simulink model "afe_dqctrl_inv_psm"  (R2026a)
settings: Solver=ode23t  StopTime=simlength  FixedStep=tc  MaxStep=glb_time.tc  RelTol=1e-4
values from neighbouring files (symbols this model uses):
  afe_ctrl = ctrl_afe_setup(glb_time.ts_afe, grid_emu.omega_grid_nom)    [init_model.m]
  afe_pwm_phase_shift_mod1 = 0    [init_model.m]
  CTRPIFF_CLIP_RELEASE = 0.001    [init_model.m]
  filters = setup_global_filters(glb_time.ts_afe, glb_time.ts_inv, glb_time.ts_dab, glb_time.tc)    [init_model.m]
  glb_time = timing_setup(fpwm_afe, trgo_afe, fpwm_inv, trgo_inv, fpwm_single_phase_inv, trgo_single_phase_inv, fpwm_dab, trgo_dab,      fpwm_psfbc, trgo_psfbc, fpwm_isop_rail, trgo_isop_rail, fpwm_cllc, trgo_cllc, t_measure, tc_factor, tc_decimation, delay_pwm, dead_time_afe,      dead_time_inv, dead_time_single_phase_inv, dead_time_dab, dead_time_psfbc, dead_time_isop_rail, dead_time_cllc)    [init_model.m]
  grid_emu = grid_three_phase_emulator('Dyn11', delta_star, grid_nominal_power, application_voltage, us1, us2, fgrid,                  eq_grid_inductance, eq_grid_resistance, eta, ucc, i1m, p_iron, n1, n2, core_area, core_length, mur,                  up_xi_pu_ref, up_eta_pu_ref, un_xi_pu_ref, un_eta_pu_ref)    [init_model.m]
  heatsink = liquid_cooled_plate_2kw_setup(weight, no_weight, cp_al, heat_capacity_hs, thermal_conductivity_al,      Rth_switch_HA, Rth_mosfet_HA, Rth_diode_HA, Tambient, DThs_init)    [init_model.m]
  inv_pwm_phase_shift_mod1 = 0    [init_model.m]
  ki_align = 18    [init_model.m]
  kp_align = 0.25    [init_model.m]
  lim_down_align = -0.05    [init_model.m]
  lim_up_align = 0.05    [init_model.m]
  omega_m_sim = psm.omega_m_bez    [init_model.m]
  psm = psm_calculus()    [init_model.m]
  psm_ctrl = ctrl_pmsm_setup(glb_time.ts_inv, psm.omega_bez, u_psm_scale, psm.Jm_norm)    [init_model.m]
  simlength = 1.75    [init_model.m]
  Tambient = 40    [init_model.m]
  time_gain_afe_module_1 = 1.0002    [init_model.m]
  time_gain_inv_module_2 = 1.001    [init_model.m]
  time_start_motor_control = 0.25    [init_model.m]
  torque_overload_factor = 1.15    [init_model.m]
  u_cm_comp_mod1 = 0    [init_model.m]
  u_psm_scale_ekf = sqrt(3)/2 * 2/3 * hwdata.inv.udc_nom/psm.ubez    [init_model.m]
undefined symbols (not defined in the file or in its folder): hwdata, igbt, magnitude, omega_m_bez, rpm_base, torque_base
libraries: fl_lib x99, nesl_utility x96, igbt_simple_lib x12, single_phase_transformer_lib x3, threephase_inductor_lib x2, dclink_for_two_levels x2, three_phase_pwm_modulator x2, cstblocks_lti x2, discrete_time_low_pass_filter x1, lithium_ion_battery x1, three_phase_voltage_with_frt_emulator x1, simple_flexible_shaft x1
(part 3 of 9)

== system afe_dqctrl_inv_psm/inv_dq_mod1/inverter/inverter ==
  gate_cmds_uvw : Inport
  sv_pwm : Subsystem
  three_phase_inverter_with_igbt_simple : Subsystem
  u : PMIOPort  Side=Left
  v : PMIOPort  Port=2  Side=Left
  w : PMIOPort  Port=3  Side=Left
  udc(+) : PMIOPort  Port=4  Side=Right
  udc(-) : PMIOPort  Port=5  Side=Right
  wires:
  sv_pwm/1(gate_cmds) -> three_phase_inverter_with_igbt_simple/1(gate_commands)
  gate_cmds_uvw/1 -> sv_pwm/1(gate_cmds_uvw)
  connections:
  three_phase_inverter_with_igbt_simple/LConn1 -- udc(+)/RConn1
  three_phase_inverter_with_igbt_simple/LConn2 -- udc(-)/RConn1
  three_phase_inverter_with_igbt_simple/RConn1 -- u/RConn1
  three_phase_inverter_with_igbt_simple/RConn2 -- v/RConn1
  three_phase_inverter_with_igbt_simple/RConn3 -- w/RConn1

== system afe_dqctrl_inv_psm/afe_dq_mod1/AFE_control/afe_control/acquisitions ==
  ug_abc_pu : Inport
  udc_pu : Inport  Port=2
  ig_abc_pu : Inport  Port=3
  is_abc_pu : Inport  Port=4
  master_time : Inport  Port=5
  grid_phase : Inport  Port=6
  Terminator : Terminator
  grid_phase_acquisition : Subsystem
  ig afe quantizzation and one step delay : Subsystem
  is afe quantizzation and one step delay : Subsystem
  phase_compensation_1 : Subsystem
  udc_acquisition : Subsystem
  ug afe quantizzation and one step delay : Subsystem
  AFE1_local_time_corr : Outport
  tag scope: grid_emulator_phase=scoped, igd_abc_pu=scoped, isd_abc_pu=scoped, udcd_pu_afe=scoped, ugd_abc_pu=scoped
  wires:
  grid_phase/1 -> grid_phase_acquisition/1(grid_phase)
  grid_phase_acquisition/1(grid_phased) -> [grid_emulator_phase]
  udc_acquisition/1(udcd_pu) -> [udcd_pu_afe]
  ig_abc_pu/1 -> ig afe quantizzation and one step delay/1(ig_abc_pu)
  ug_abc_pu/1 -> ug afe quantizzation and one step delay/1(ug_abc_pu)
  [udcd_pu_afe] -> Terminator/1
  phase_compensation_1/1(y) -> AFE1_local_time_corr/1
  is_abc_pu/1 -> is afe quantizzation and one step delay/1(is_abc_pu)
  master_time/1 -> phase_compensation_1/2(master_time)
  udc_pu/1 -> udc_acquisition/1(udc_pu)
  ig afe quantizzation and one step delay/1(igd_abc_pu) -> [igd_abc_pu]
  [local_time] -> phase_compensation_1/1(local_time)
  is afe quantizzation and one step delay/1(isd_abc_pu) -> [isd_abc_pu]
  ug afe quantizzation and one step delay/1(ugd_abc_pu) -> [ugd_abc_pu]

== system afe_dqctrl_inv_psm/afe_dq_mod1/AFE_control/afe_control/current_ctrl ==
  i_xi_ref : Inport
  Constant : Constant  Value=0
  Demux : Demux  Outputs=3
  current_transformation : Subsystem
  dq_vector_pi : Subsystem
  xi_eta_to_alpha_beta : MATLAB Function  TreatAsAtomicUnit=on
  zero_current_ctrl : Subsystem
  uabg : Outport  VectorParamsAs1DForOutWhenUnconnected=off
  wires:
  Demux/1 -> current_transformation/1(is_a_pu)  "is_a"
  Demux/2 -> current_transformation/2(is_b_pu)  "is_b"
  Demux/3 -> current_transformation/3(is_c_pu)  "is_c"
  [isd_abc_pu] -> Demux/1
  [phase_grid_pll] -> xi_eta_to_alpha_beta/3(phase)
  [id_xi_pu] -> dq_vector_pi/1(id)
  [id_eta_pu] -> dq_vector_pi/3(iq)
  i_xi_ref/1 -> dq_vector_pi/2(id_ref)
  Constant/1 -> dq_vector_pi/4(iq_ref)
  zero_current_ctrl/1(uabg_ctrl_out) -> uabg/1
  dq_vector_pi/1(md_sat) -> xi_eta_to_alpha_beta/1(xi)
  dq_vector_pi/2(mq_sat) -> xi_eta_to_alpha_beta/2(eta)
  xi_eta_to_alpha_beta/1(alpha) -> zero_current_ctrl/1(ualpha_ctrl_afe)
  xi_eta_to_alpha_beta/2(beta) -> zero_current_ctrl/2(ubeta_ctrl_afe)

== system afe_dqctrl_inv_psm/afe_dq_mod1/AFE_control/afe_control/data_to_worspace_module_1 ==
  Bus Creator : BusCreator  Inputs=3
  dq_pll : Subsystem
  pwr_meter : Subsystem
  m : Outport
  wires:
  Bus Creator/1 -> m/1
  pwr_meter/1(m_pwr_meter) -> Bus Creator/1  "pwr_meter"
  dq_pll/1(dqPLLs) -> Bus Creator/2  "dq_pll"
  [local_time] -> Bus Creator/3  "local_time"

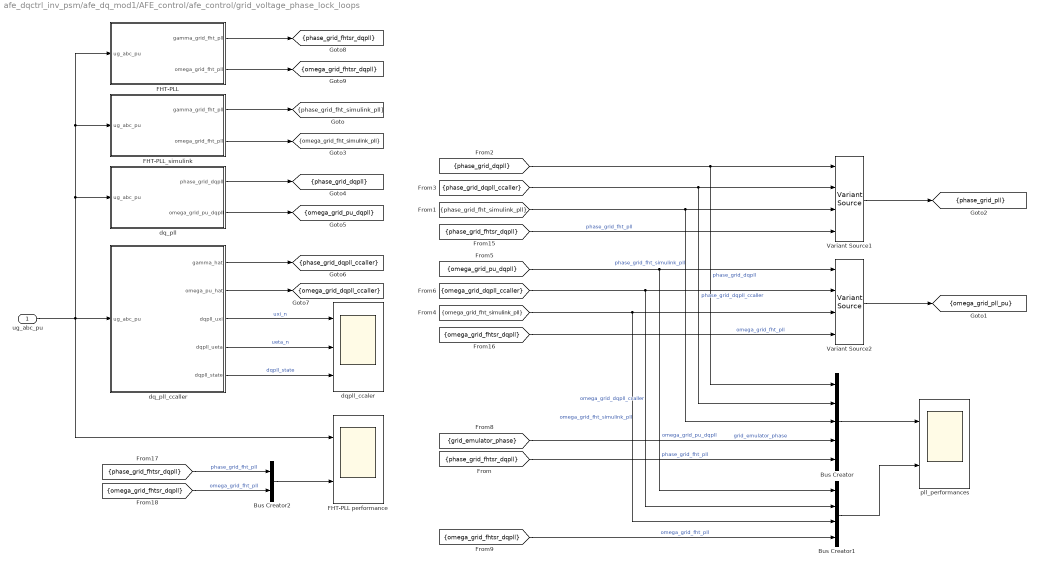
== system afe_dqctrl_inv_psm/afe_dq_mod1/AFE_control/afe_control/grid_voltage_phase_lock_loops ==
  ug_abc_pu : Inport
  Bus Creator : BusCreator  Inputs=5
  Bus Creator1 : BusCreator  Inputs=4
  Bus Creator2 : BusCreator  Inputs=2
  FHT-PLL : Subsystem
  FHT-PLL performance : Scope  NumInputPorts=2
      settings: ActiveDisplayYMinimum=-1.251220703125  ActiveDisplayYMaximum=1.251220703125  DataLoggingVariableName=ScopeData8
  FHT-PLL_simulink : Subsystem
  Variant Source1 : VariantSource  VariantControls={use_dq_pll_mode1 == 1, use_dq_pll_mode2 == 1, use_dq_pll_mode3 == 1, use_dq_pll_mode4 == 1}
  Variant Source2 : VariantSource  VariantControls={use_dq_pll_mode1 == 1, use_dq_pll_mode2 == 1, use_dq_pll_mode3 == 1, use_dq_pll_mode4 == 1}
  dq_pll : Subsystem
  dq_pll_ccaller : Subsystem
  dqpll_ccaler : Scope  NumInputPorts=3
      settings: ActiveDisplayYMinimum=-0.88802937790751446  ActiveDisplayYMaximum=4.5431143753230572  DataLoggingVariableName=ScopeData4
  pll_performances : Scope  NumInputPorts=2
      settings: ActiveDisplayYMinimum=-3.9264641704366507  ActiveDisplayYMaximum=3.9264746341683896  DataLoggingVariableName=ScopeData34
  tag scope: omega_grid_dqpll_ccaller=scoped, omega_grid_fht_simulink_pll=scoped, omega_grid_fhtsr_dqpll=scoped, omega_grid_pll_pu=scoped, omega_grid_pu_dqpll=scoped, phase_grid_dqpll=scoped, phase_grid_dqpll_ccaller=scoped, phase_grid_fht_simulink_pll=scoped, phase_grid_fhtsr_dqpll=scoped, phase_grid_pll=scoped
  wires:
  Variant Source1/1 -> [phase_grid_pll]
  FHT-PLL_simulink/1(gamma_grid_fht_pll) -> [phase_grid_fht_simulink_pll]
  FHT-PLL_simulink/2(omega_grid_fht_pll) -> [omega_grid_fht_simulink_pll]
  dq_pll/2(omega_grid_pu_dqpll) -> [omega_grid_pu_dqpll]
  dq_pll/1(phase_grid_dqpll) -> [phase_grid_dqpll]
  dq_pll_ccaller/1(gamma_hat) -> [phase_grid_dqpll_ccaller]
  dq_pll_ccaller/2(omega_pu_hat) -> [omega_grid_dqpll_ccaller]
  [phase_grid_dqpll] -> Variant Source1/1, Bus Creator/1  "phase_grid_dqpll"
  [phase_grid_dqpll_ccaller] -> Bus Creator/2, Variant Source1/2  "phase_grid_dqpll_ccaller"
  [phase_grid_fht_simulink_pll] -> Bus Creator/3, Variant Source1/3  "phase_grid_fht_simulink_pll"
  [omega_grid_pu_dqpll] -> Variant Source2/1, Bus Creator1/1  "omega_grid_pu_dqpll"
  [omega_grid_dqpll_ccaller] -> Variant Source2/2, Bus Creator1/2  "omega_grid_dqpll_ccaller"
  [omega_grid_fht_simulink_pll] -> Variant Source2/3, Bus Creator1/3  "omega_grid_fht_simulink_pll"
  Variant Source2/1 -> [omega_grid_pll_pu]
  dq_pll_ccaller/3(dqpll_uxi) -> dqpll_ccaler/1  "uxi_n"
  dq_pll_ccaller/4(dqpll_ueta) -> dqpll_ccaler/2  "ueta_n"
  dq_pll_ccaller/5(dqpll_state) -> dqpll_ccaler/3  "dqpll_state"
  ug_abc_pu/1 -> FHT-PLL performance/1, dq_pll/1(ug_abc_pu), FHT-PLL_simulink/1(ug_abc_pu), FHT-PLL/1(ug_abc_pu), dq_pll_ccaller/1(ug_abc_pu)
  Bus Creator/1 -> pll_performances/1
  Bus Creator1/1 -> pll_performances/2
  [grid_emulator_phase] -> Bus Creator/4  "grid_emulator_phase"
  FHT-PLL/2(omega_grid_fht_pll) -> [omega_grid_fhtsr_dqpll]
  FHT-PLL/1(gamma_grid_fht_pll) -> [phase_grid_fhtsr_dqpll]
  [phase_grid_fhtsr_dqpll] -> Bus Creator/5  "phase_grid_fht_pll"
  [omega_grid_fhtsr_dqpll] -> Bus Creator1/4  "omega_grid_fht_pll"
  [phase_grid_fhtsr_dqpll] -> Variant Source1/4  "phase_grid_fht_pll"
  [omega_grid_fhtsr_dqpll] -> Variant Source2/4  "omega_grid_fht_pll"
  Bus Creator2/1 -> FHT-PLL performance/2
  [omega_grid_fhtsr_dqpll] -> Bus Creator2/2  "omega_grid_fht_pll"
  [phase_grid_fhtsr_dqpll] -> Bus Creator2/1  "phase_grid_fht_pll"

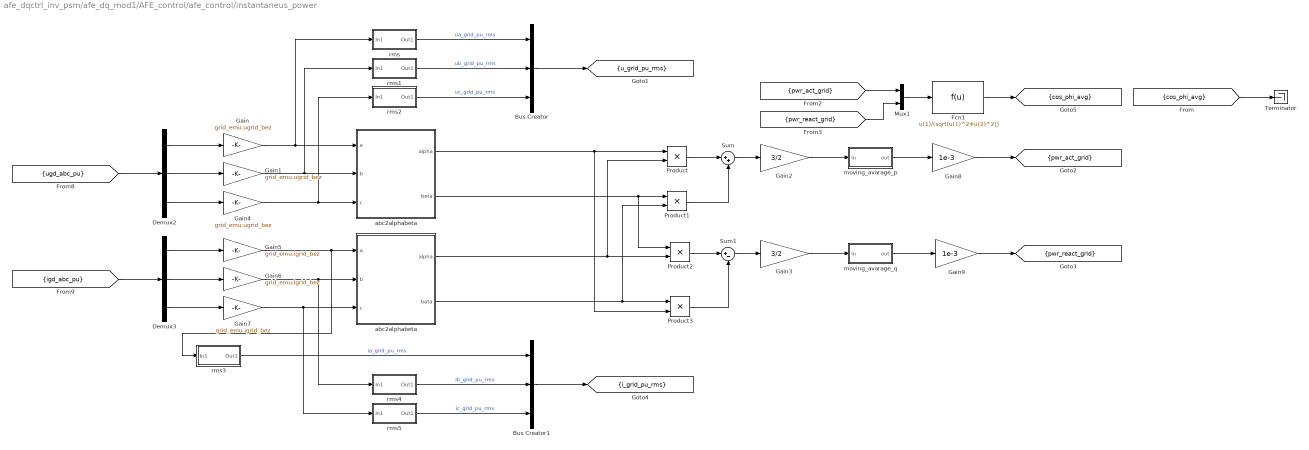
== system afe_dqctrl_inv_psm/afe_dq_mod1/AFE_control/afe_control/instantaneus_power ==
  Bus Creator : BusCreator  Inputs=3
  Bus Creator1 : BusCreator  Inputs=3
  Demux2 : Demux  Outputs=3
  Demux3 : Demux  Outputs=3
  Fcn1 : Fcn  Expr=u(1)/(sqrt(u(1)^2+u(2)^2))
  Gain : Gain  Gain=grid_emu.ugrid_bez
  Gain1 : Gain  Gain=grid_emu.ugrid_bez
  Gain2 : Gain  Gain=3/2
  Gain3 : Gain  Gain=3/2
  Gain4 : Gain  Gain=grid_emu.ugrid_bez
  Gain5 : Gain  Gain=grid_emu.igrid_bez
  Gain6 : Gain  Gain=grid_emu.igrid_bez
  Gain7 : Gain  Gain=grid_emu.igrid_bez
  Gain8 : Gain  Gain=1e-3
  Gain9 : Gain  Gain=1e-3
  Mux1 : Mux  Inputs=2
  Product{,1..3} (4 alike) : Product  RndMeth=Zero
  Sum : Sum  Inputs=|++
  Sum1 : Sum  Inputs=|+-
  Terminator : Terminator
  abc2alphabeta : Subsystem
  "abc2alphabeta " : Subsystem
  moving_avarage_p : Subsystem
  moving_avarage_q : Subsystem
  rms : Subsystem
  rms1 : Subsystem
  rms2 : Subsystem
  rms3 : Subsystem
  rms4 : Subsystem
  rms5 : Subsystem
  tag scope: cos_phi_avg=scoped, i_grid_pu_rms=scoped, pwr_act_grid=scoped, pwr_react_grid=scoped, u_grid_pu_rms=scoped
  wires:
  abc2alphabeta/2("beta ") -> Product1/1, Product2/1
  "abc2alphabeta "/2("beta ") -> Product1/2, Product3/1
  abc2alphabeta/1("alpha ") -> Product3/2, Product/1
  "abc2alphabeta "/1("alpha ") -> Product2/2, Product/2
  Product/1 -> Sum/1
  Product1/1 -> Sum/2
  Product2/1 -> Sum1/1
  Product3/1 -> Sum1/2
  Sum1/1 -> Gain3/1
  Sum/1 -> Gain2/1
  Gain2/1 -> moving_avarage_p/1(in)
  Gain3/1 -> moving_avarage_q/1(in)
  [pwr_react_grid] -> Mux1/2
  Mux1/1 -> Fcn1/1
  Fcn1/1 -> [cos_phi_avg]
  [pwr_act_grid] -> Mux1/1
  rms/1(Out1) -> Bus Creator/1  "ua_grid_pu_rms"
  rms2/1(Out1) -> Bus Creator/3  "uc_grid_pu_rms"
  rms1/1(Out1) -> Bus Creator/2  "ub_grid_pu_rms"
  moving_avarage_p/1(out) -> Gain8/1
  moving_avarage_q/1(out) -> Gain9/1
  Demux2/1 -> Gain/1
  Demux2/2 -> Gain1/1
  Demux2/3 -> Gain4/1
  Demux3/1 -> Gain5/1
  Demux3/2 -> Gain6/1
  Demux3/3 -> Gain7/1
  Gain/1 -> rms/1(In1), abc2alphabeta/1(a)
  Gain1/1 -> rms1/1(In1), abc2alphabeta/2(b)
  Gain4/1 -> rms2/1(In1), abc2alphabeta/3(c)
  Gain5/1 -> rms3/1(In1), "abc2alphabeta "/1(a)
  Gain6/1 -> rms4/1(In1), "abc2alphabeta "/2(b)
  Gain7/1 -> rms5/1(In1), "abc2alphabeta "/3(c)
  Gain8/1 -> [pwr_act_grid]
  Gain9/1 -> [pwr_react_grid]
  [ugd_abc_pu] -> Demux2/1
  [igd_abc_pu] -> Demux3/1
  Bus Creator/1 -> [u_grid_pu_rms]
  rms4/1(Out1) -> Bus Creator1/2  "ib_grid_pu_rms"
  rms3/1(Out1) -> Bus Creator1/1  "ia_grid_pu_rms"
  rms5/1(Out1) -> Bus Creator1/3  "ic_grid_pu_rms"
  Bus Creator1/1 -> [i_grid_pu_rms]
  [cos_phi_avg] -> Terminator/1

== system afe_dqctrl_inv_psm/afe_dq_mod1/AFE_control/afe_control/interesting scopes ==
  current_sequences_mod1 : Scope  NumInputPorts=4
      settings: ActiveDisplayYMinimum=-0.97178065031766891  ActiveDisplayYMaximum=1.9392475411295891  DataLoggingVariableName=ScopeData2
  i_grid_seq_ref : Scope
      settings: ActiveDisplayYMinimum=-1.1499999999999995  ActiveDisplayYMaximum=0.34999999999999981
  voltage_sequences_mod1 : Scope  NumInputPorts=4
      settings: ActiveDisplayYMinimum=-1.2405151816982258  ActiveDisplayYMaximum=1.2605257614333911
  wires:
  [v_grid_neg_eta_avg] -> voltage_sequences_mod1/4  "u_grid_neg_eta"
  [i_grid_neg_xi_avg] -> current_sequences_mod1/3  "i_grid_neg_xi"
  [v_grid_pos_eta_avg] -> voltage_sequences_mod1/2  "u_grid_pos_eta"
  [v_grid_neg_xi_avg] -> voltage_sequences_mod1/3  "u_grid_neg_xi"
  [i_grid_pos_xi_avg] -> current_sequences_mod1/1  "i_grid_pos_xi"
  [i_grid_neg_eta_avg] -> current_sequences_mod1/4  "i_grid_neg_eta"
  [v_grid_pos_xi_avg] -> voltage_sequences_mod1/1  "u_grid_pos_xi"
  [i_grid_pos_eta_avg] -> current_sequences_mod1/2  "i_grid_pos_eta"
  [i_grid_seq_ref] -> i_grid_seq_ref/1  "i_grid_seq_ref"

== system afe_dqctrl_inv_psm/afe_dq_mod1/AFE_control/afe_control/space_vector ==
  uab_out : Inport
  Bus Creator : BusCreator  Inputs=3
  Bus Selector : BusSelector  OutputSignals=da,db,dc
  Bus Selector1 : BusSelector  OutputSignals=ualpha_ctrl_afe,ubeta_ctrl_afe,ugamma_ctrl_afe
  C Caller : CCaller  FunctionName=sv_pwm_cm_process_simulink  PortSpecificationStruct="%)30     .    B H   8    (     @         %    \"     8    !     0         %  0 \"0    $    _    07)G3F%M90  4&]R=$YA;64 4V-O<&4     26YD97@     5'EP90      4VEZ90      27-';&]B86P   X    P    !@    @    $          4    (     0    ,    !         !   P!O=70 #@   #     &    \"     0         !0    @    !     P    $         $  # &]U=  .    .     8    (    !          %    \"     $    &     0         0   ...(+3252 chars)"
  Constant : Constant  Value=glb_time.ts_afe
  Constant1 : Constant
  Data Type Conversion1 : DataTypeConversion  OutDataTypeStr=double  SaturateOnIntegerOverflow=off  RndMeth=Floor
  Data Type Conversion{4,15..16,18} (4 alike) : DataTypeConversion  OutDataTypeStr=single  SaturateOnIntegerOverflow=off  RndMeth=Floor
  Data Type Conversion17 : DataTypeConversion  OutDataTypeStr=uint32  SaturateOnIntegerOverflow=off  RndMeth=Floor
  Data Type Conversion2 : DataTypeConversion  OutDataTypeStr=double  SaturateOnIntegerOverflow=off  RndMeth=Floor
  Data Type Conversion3 : DataTypeConversion  OutDataTypeStr=double  SaturateOnIntegerOverflow=off  RndMeth=Floor
  Gain1 : Gain  Gain=sqrt(3)/2
  Gain2 : Gain  Gain=sqrt(3)/2
  Gain3 : Gain  Gain=u_cm_comp_mod1
  duvw : Outport
  wires:
  Data Type Conversion15/1 -> C Caller/2
  Bus Selector/2 -> Data Type Conversion2/1  "<db>"
  Data Type Conversion18/1 -> C Caller/1
  C Caller/1 -> Bus Selector/1
  Bus Creator/1 -> duvw/1
  Data Type Conversion1/1 -> Bus Creator/1  "du(k)"
  Bus Selector1/2 -> Gain2/1  "<ubeta_ctrl_afe>"
  Bus Selector/3 -> Data Type Conversion3/1  "<dc>"
  Bus Selector1/1 -> Gain1/1  "<ualpha_ctrl_afe>"
  Data Type Conversion2/1 -> Bus Creator/2  "dv(k)"
  Gain2/1 -> Data Type Conversion15/1
  Bus Selector/1 -> Data Type Conversion1/1  "<da>"
  Gain1/1 -> Data Type Conversion18/1
  Data Type Conversion3/1 -> Bus Creator/3  "dw(k)"
  Constant/1 -> Data Type Conversion16/1
  uab_out/1 -> Bus Selector1/1
  Constant1/1 -> Data Type Conversion17/1
  Data Type Conversion16/1 -> C Caller/4
  Data Type Conversion17/1 -> C Caller/5
  Bus Selector1/3 -> Gain3/1  "<ugamma_ctrl_afe>"
  Gain3/1 -> Data Type Conversion4/1
  Data Type Conversion4/1 -> C Caller/3

== system afe_dqctrl_inv_psm/afe_dq_mod1/AFE_control/afe_control/udc_ctrl ==
  udc_pu : Inport
  1/Ti : Gain  Gain=afe_ctrl.kp_udc_ctrl  SaturateOnIntegerOverflow=on  OutDataTypeStr=Inherit: Same as input  ParamDataTypeStr=Inherit: Same as input
  Constant : Constant  Value=0
  Gain : Gain  Gain=-1
  Saturation : Saturate  UpperLimit=afe_ctrl.ixi_pos_ref_lim  LowerLimit=-afe_ctrl.ixi_pos_ref_lim
  Sum1 : Sum  Inputs=+++  SaturateOnIntegerOverflow=on
  Sum2 : Sum  Inputs=-+  SaturateOnIntegerOverflow=on
  Sum3 : Sum  Inputs=-+  SaturateOnIntegerOverflow=on
  Switch : Switch  Criteria=u2 > Threshold  SaturateOnIntegerOverflow=off  InputSameDT=off
  To Workspace1 : ToWorkspace  VariableName=udc_pu_sim_mod1  SampleTime=-1
      settings: MaxDataPoints=glb_time.Ns_afe
  To Workspace3 : ToWorkspace  VariableName=udc_pu_ref_sim_mod1  SampleTime=-1
      settings: MaxDataPoints=glb_time.Ns_afe
  Unit Delay4 : UnitDelay  SampleTime=-1
  discrete-time-low-pass-filter1 : discrete_time_low_pass_filter/discrete-time-low-pass-filter  tau=20e-3  ts=glb_time.ts_afe
  kp : Gain  Gain=afe_ctrl.ki_udc_ctrl*glb_time.ts_afe  SaturateOnIntegerOverflow=on  OutDataTypeStr=Inherit: Same as input  ParamDataTypeStr=Inherit: Same as input
  udc_norm_ref : Step  Time=1e-3  FinalValue=afe_ctrl.udc_norm_ref
  udc_tracking : Scope  NumInputPorts=3
      settings: ActiveDisplayYMinimum=-2.0004150390624997  ActiveDisplayYMaximum=1.5037353515624998  DataLoggingVariableName=ScopeData8
  i_xi_ref : Outport
  wires:
  1/Ti/1 -> Sum1/1, Sum3/1
  kp/1 -> Sum1/2
  Sum3/1 -> Unit Delay4/1
  Unit Delay4/1 -> Sum1/3
  udc_norm_ref/1 -> discrete-time-low-pass-filter1/1
  udc_pu/1 -> Sum2/1, To Workspace1/1, udc_tracking/2  "udc_pu"
  Sum2/1 -> kp/1, 1/Ti/1
  Sum1/1 -> Saturation/1
  [pwr_lim_enable] -> Switch/2
  Saturation/1 -> Switch/3
  Switch/1 -> Sum3/2, Gain/1
  Constant/1 -> Switch/1
  Gain/1 -> udc_tracking/3, i_xi_ref/1  "i_xi_ref"
  discrete-time-low-pass-filter1/1 -> To Workspace3/1, udc_tracking/1, Sum2/2  "udc_pu_ref"

== system afe_dqctrl_inv_psm/afe_dq_mod1/afe/sv_pwm/modulator1 ==
  u : Inport
  v : Inport  Port=2
  w : Inport  Port=3
  phase : Inport  Port=4
  Bus Creator : BusCreator  Inputs=3
  Three phase two level PWM generator with global TRGO : three_phase_pwm_modulator/Three phase two level PWM generator with global TRGO  f=glb_time.fPWM_AFE  m_up=0.98  m_low=0.02  dead_time=glb_time.dead_time_AFE  pos_cmd_gate=15  neg_cmd_gate=-10  polarity=1  tc=glb_time.tc  double_sampling=glb_time.TRGO_AFE_double_update
      link override gate commands/Bus Selector: OutputSignals=du(t)
      link override gate commands/Bus Selector1: OutputSignals=dv(t)
      link override gate commands/Bus Selector2: OutputSignals=dw(t)
  gate_cmds : Outport
  tag scope: TRGO_afe_module_1=global
  wires:
  Bus Creator/1 -> Three phase two level PWM generator with global TRGO/3
  Three phase two level PWM generator with global TRGO/1 -> [TRGO_afe_module_1]
  u/1 -> Bus Creator/1
  v/1 -> Bus Creator/2
  w/1 -> Bus Creator/3
  phase/1 -> Three phase two level PWM generator with global TRGO/2
  Three phase two level PWM generator with global TRGO/2 -> gate_cmds/1
  [time_afe_module_1] -> Three phase two level PWM generator with global TRGO/1

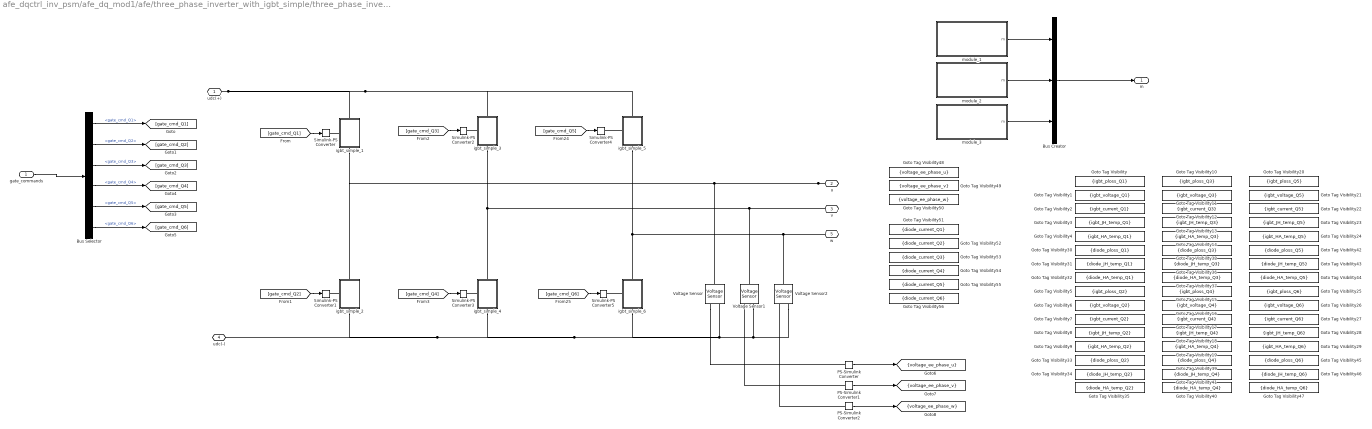
== system afe_dqctrl_inv_psm/afe_dq_mod1/afe/three_phase_inverter_with_igbt_simple/three_phase_inverter_with_igbt_simple ==
  gate_commands : Inport
  Bus Creator : BusCreator  Inputs=3
  Bus Selector : BusSelector  OutputSignals=gate_cmd_Q1,gate_cmd_Q2,gate_cmd_Q3,gate_cmd_Q4,gate_cmd_Q5,gate_cmd_Q6
  Goto Tag Visibility : GotoTagVisibility  GotoTag=igbt_ploss_Q1
  Goto Tag Visibility1 : GotoTagVisibility  GotoTag=igbt_voltage_Q1
  Goto Tag Visibility10 : GotoTagVisibility  GotoTag=igbt_ploss_Q3
  Goto Tag Visibility11 : GotoTagVisibility  GotoTag=igbt_voltage_Q3
  Goto Tag Visibility12 : GotoTagVisibility  GotoTag=igbt_current_Q3
  Goto Tag Visibility13 : GotoTagVisibility  GotoTag=igbt_JH_temp_Q3
  Goto Tag Visibility14 : GotoTagVisibility  GotoTag=igbt_HA_temp_Q3
  Goto Tag Visibility15 : GotoTagVisibility  GotoTag=igbt_ploss_Q4
  Goto Tag Visibility16 : GotoTagVisibility  GotoTag=igbt_voltage_Q4
  Goto Tag Visibility17 : GotoTagVisibility  GotoTag=igbt_current_Q4
  Goto Tag Visibility18 : GotoTagVisibility  GotoTag=igbt_JH_temp_Q4
  Goto Tag Visibility19 : GotoTagVisibility  GotoTag=igbt_HA_temp_Q4
  Goto Tag Visibility2 : GotoTagVisibility  GotoTag=igbt_current_Q1
  Goto Tag Visibility20 : GotoTagVisibility  GotoTag=igbt_ploss_Q5
  Goto Tag Visibility21 : GotoTagVisibility  GotoTag=igbt_voltage_Q5
  Goto Tag Visibility22 : GotoTagVisibility  GotoTag=igbt_current_Q5
  Goto Tag Visibility23 : GotoTagVisibility  GotoTag=igbt_JH_temp_Q5
  Goto Tag Visibility24 : GotoTagVisibility  GotoTag=igbt_HA_temp_Q5
  Goto Tag Visibility25 : GotoTagVisibility  GotoTag=igbt_ploss_Q6
  Goto Tag Visibility26 : GotoTagVisibility  GotoTag=igbt_voltage_Q6
  Goto Tag Visibility27 : GotoTagVisibility  GotoTag=igbt_current_Q6
  Goto Tag Visibility28 : GotoTagVisibility  GotoTag=igbt_JH_temp_Q6
  Goto Tag Visibility29 : GotoTagVisibility  GotoTag=igbt_HA_temp_Q6
  Goto Tag Visibility3 : GotoTagVisibility  GotoTag=igbt_JH_temp_Q1
  Goto Tag Visibility30 : GotoTagVisibility  GotoTag=diode_ploss_Q1
  Goto Tag Visibility31 : GotoTagVisibility  GotoTag=diode_JH_temp_Q1
  Goto Tag Visibility32 : GotoTagVisibility  GotoTag=diode_HA_temp_Q1
  Goto Tag Visibility33 : GotoTagVisibility  GotoTag=diode_ploss_Q2
  Goto Tag Visibility34 : GotoTagVisibility  GotoTag=diode_JH_temp_Q2
  Goto Tag Visibility35 : GotoTagVisibility  GotoTag=diode_HA_temp_Q2
  Goto Tag Visibility36 : GotoTagVisibility  GotoTag=diode_JH_temp_Q3
  Goto Tag Visibility37 : GotoTagVisibility  GotoTag=diode_HA_temp_Q3
  Goto Tag Visibility38 : GotoTagVisibility  GotoTag=diode_ploss_Q3
  Goto Tag Visibility39 : GotoTagVisibility  GotoTag=diode_ploss_Q4
  Goto Tag Visibility4 : GotoTagVisibility  GotoTag=igbt_HA_temp_Q1
  Goto Tag Visibility40 : GotoTagVisibility  GotoTag=diode_HA_temp_Q4
  Goto Tag Visibility41 : GotoTagVisibility  GotoTag=diode_JH_temp_Q4
  Goto Tag Visibility42 : GotoTagVisibility  GotoTag=diode_ploss_Q5
  Goto Tag Visibility43 : GotoTagVisibility  GotoTag=diode_JH_temp_Q5
  Goto Tag Visibility44 : GotoTagVisibility  GotoTag=diode_HA_temp_Q5
  Goto Tag Visibility45 : GotoTagVisibility  GotoTag=diode_ploss_Q6
  Goto Tag Visibility46 : GotoTagVisibility  GotoTag=diode_JH_temp_Q6
  Goto Tag Visibility47 : GotoTagVisibility  GotoTag=diode_HA_temp_Q6
  Goto Tag Visibility48 : GotoTagVisibility  GotoTag=voltage_ee_phase_u
  Goto Tag Visibility49 : GotoTagVisibility  GotoTag=voltage_ee_phase_v
  Goto Tag Visibility5 : GotoTagVisibility  GotoTag=igbt_ploss_Q2
  Goto Tag Visibility50 : GotoTagVisibility  GotoTag=voltage_ee_phase_w
  Goto Tag Visibility51 : GotoTagVisibility  GotoTag=diode_current_Q1
  Goto Tag Visibility52 : GotoTagVisibility  GotoTag=diode_current_Q2
  Goto Tag Visibility53 : GotoTagVisibility  GotoTag=diode_current_Q3
  Goto Tag Visibility54 : GotoTagVisibility  GotoTag=diode_current_Q4
  Goto Tag Visibility55 : GotoTagVisibility  GotoTag=diode_current_Q5
  Goto Tag Visibility56 : GotoTagVisibility  GotoTag=diode_current_Q6
  Goto Tag Visibility6 : GotoTagVisibility  GotoTag=igbt_voltage_Q2
  Goto Tag Visibility7 : GotoTagVisibility  GotoTag=igbt_current_Q2
  Goto Tag Visibility8 : GotoTagVisibility  GotoTag=igbt_JH_temp_Q2
  Goto Tag Visibility9 : GotoTagVisibility  GotoTag=igbt_HA_temp_Q2
  PS-Simulink Converter : nesl_utility/PS-Simulink Converter  PhysicalDomain=network_engine_domain  SubClassName=ps_output  LeftPortType=input  RightPortType=output  PseudoPeriodic=off  Frequencies=[]  VectorFormat=1-D array  Unit=V  AffineConversion=off
  PS-Simulink Converter1 : nesl_utility/PS-Simulink Converter  PhysicalDomain=network_engine_domain  SubClassName=ps_output  LeftPortType=input  RightPortType=output  PseudoPeriodic=off  Frequencies=[]  VectorFormat=1-D array  Unit=V  AffineConversion=off
  PS-Simulink Converter2 : nesl_utility/PS-Simulink Converter  PhysicalDomain=network_engine_domain  SubClassName=ps_output  LeftPortType=input  RightPortType=output  PseudoPeriodic=off  Frequencies=[]  VectorFormat=1-D array  Unit=V  AffineConversion=off
  Simulink-PS Converter{,1..5} (6 alike) : nesl_utility/Simulink-PS Converter  PhysicalDomain=network_engine_domain  SubClassName=ps_input  LeftPortType=input  RightPortType=output  PseudoPeriodic=off  Frequencies=[]  NoiseDistribution=none  NoiseParameters=[]  Unit=V  AffineConversion=off  FilteringAndDerivatives=provide  SimscapeFilterOrder=1  InputFilterTimeConstant=0.001  UdotUserProvided=0
  Voltage Sensor : fl_lib/Electrical/Electrical Sensors/Voltage Sensor
  Voltage Sensor1 : fl_lib/Electrical/Electrical Sensors/Voltage Sensor
  Voltage Sensor2 : fl_lib/Electrical/Electrical Sensors/Voltage Sensor
  igbt_simple_1 : Subsystem
      settings: PortSchema="{\"entries\":[{\"content\":{\"sides\":[{\"content\":{\"connectorIds\":[\"LConn1\"]},\"type\":\"ConnectorPlacement.EquallySpacedRectSide\",\"uuid\":\"9277da8d-d460-43e6-8478-dd662f15d226\"},{\"content\":{\"connectorIds\":[],\"side\":\"RIGHT\"},\"type\":\"ConnectorPlacement.EquallySpacedRectSide\",\"uuid\":\"a7ece396-f1d9-4f4f-a05b-db1fc65d6e1d\"},{\"content\":{\"connectorIds\":[\"LConn2\"],\"side\":\"TOP\"},\"type\":\"ConnectorPlacement.EquallySpacedRectSide\",\"uuid\":\"fdd70777-e9cf-4317-afb6-cae87f75d5b0\"},{\"content\":{\"connectorIds\":[\"RConn1\"],\"side\":\"BOTTOM\"},\"type\":\"ConnectorPlacement.EquallySpacedRectSide\",\"uuid\":\"2353ed68-b1a1-4775-9ca9-31e268d5443b\"}]},\"type\":\"ConnectorPlacement.EquallySpacedConnector\",\"uuid\":\"d5479f4c-4e65-4791-adcb-73df11f88590\"}],\"packageUris\":[\"http://schema.mathworks.com/mf0/Connector/R2020b\"],\"version\":\"1.0\"}"
  igbt_simple_2 : Subsystem
      settings: PortSchema="{\"entries\":[{\"content\":{\"sides\":[{\"content\":{\"connectorIds\":[\"LConn1\"]},\"type\":\"ConnectorPlacement.EquallySpacedRectSide\",\"uuid\":\"9277da8d-d460-43e6-8478-dd662f15d226\"},{\"content\":{\"connectorIds\":[],\"side\":\"RIGHT\"},\"type\":\"ConnectorPlacement.EquallySpacedRectSide\",\"uuid\":\"a7ece396-f1d9-4f4f-a05b-db1fc65d6e1d\"},{\"content\":{\"connectorIds\":[\"LConn2\"],\"side\":\"TOP\"},\"type\":\"ConnectorPlacement.EquallySpacedRectSide\",\"uuid\":\"fdd70777-e9cf-4317-afb6-cae87f75d5b0\"},{\"content\":{\"connectorIds\":[\"RConn1\"],\"side\":\"BOTTOM\"},\"type\":\"ConnectorPlacement.EquallySpacedRectSide\",\"uuid\":\"2353ed68-b1a1-4775-9ca9-31e268d5443b\"}]},\"type\":\"ConnectorPlacement.EquallySpacedConnector\",\"uuid\":\"d5479f4c-4e65-4791-adcb-73df11f88590\"}],\"packageUris\":[\"http://schema.mathworks.com/mf0/Connector/R2020b\"],\"version\":\"1.0\"}"
  igbt_simple_3 : Subsystem
      settings: PortSchema="{\"entries\":[{\"content\":{\"sides\":[{\"content\":{\"connectorIds\":[\"LConn1\"]},\"type\":\"ConnectorPlacement.EquallySpacedRectSide\",\"uuid\":\"9277da8d-d460-43e6-8478-dd662f15d226\"},{\"content\":{\"connectorIds\":[],\"side\":\"RIGHT\"},\"type\":\"ConnectorPlacement.EquallySpacedRectSide\",\"uuid\":\"a7ece396-f1d9-4f4f-a05b-db1fc65d6e1d\"},{\"content\":{\"connectorIds\":[\"LConn2\"],\"side\":\"TOP\"},\"type\":\"ConnectorPlacement.EquallySpacedRectSide\",\"uuid\":\"fdd70777-e9cf-4317-afb6-cae87f75d5b0\"},{\"content\":{\"connectorIds\":[\"RConn1\"],\"side\":\"BOTTOM\"},\"type\":\"ConnectorPlacement.EquallySpacedRectSide\",\"uuid\":\"2353ed68-b1a1-4775-9ca9-31e268d5443b\"}]},\"type\":\"ConnectorPlacement.EquallySpacedConnector\",\"uuid\":\"d5479f4c-4e65-4791-adcb-73df11f88590\"}],\"packageUris\":[\"http://schema.mathworks.com/mf0/Connector/R2020b\"],\"version\":\"1.0\"}"
  igbt_simple_4 : Subsystem
      settings: PortSchema="{\"entries\":[{\"content\":{\"sides\":[{\"content\":{\"connectorIds\":[\"LConn1\"]},\"type\":\"ConnectorPlacement.EquallySpacedRectSide\",\"uuid\":\"9277da8d-d460-43e6-8478-dd662f15d226\"},{\"content\":{\"connectorIds\":[],\"side\":\"RIGHT\"},\"type\":\"ConnectorPlacement.EquallySpacedRectSide\",\"uuid\":\"a7ece396-f1d9-4f4f-a05b-db1fc65d6e1d\"},{\"content\":{\"connectorIds\":[\"LConn2\"],\"side\":\"TOP\"},\"type\":\"ConnectorPlacement.EquallySpacedRectSide\",\"uuid\":\"fdd70777-e9cf-4317-afb6-cae87f75d5b0\"},{\"content\":{\"connectorIds\":[\"RConn1\"],\"side\":\"BOTTOM\"},\"type\":\"ConnectorPlacement.EquallySpacedRectSide\",\"uuid\":\"2353ed68-b1a1-4775-9ca9-31e268d5443b\"}]},\"type\":\"ConnectorPlacement.EquallySpacedConnector\",\"uuid\":\"d5479f4c-4e65-4791-adcb-73df11f88590\"}],\"packageUris\":[\"http://schema.mathworks.com/mf0/Connector/R2020b\"],\"version\":\"1.0\"}"
  igbt_simple_5 : Subsystem
      settings: PortSchema="{\"entries\":[{\"content\":{\"sides\":[{\"content\":{\"connectorIds\":[\"LConn1\"]},\"type\":\"ConnectorPlacement.EquallySpacedRectSide\",\"uuid\":\"9277da8d-d460-43e6-8478-dd662f15d226\"},{\"content\":{\"connectorIds\":[],\"side\":\"RIGHT\"},\"type\":\"ConnectorPlacement.EquallySpacedRectSide\",\"uuid\":\"a7ece396-f1d9-4f4f-a05b-db1fc65d6e1d\"},{\"content\":{\"connectorIds\":[\"LConn2\"],\"side\":\"TOP\"},\"type\":\"ConnectorPlacement.EquallySpacedRectSide\",\"uuid\":\"fdd70777-e9cf-4317-afb6-cae87f75d5b0\"},{\"content\":{\"connectorIds\":[\"RConn1\"],\"side\":\"BOTTOM\"},\"type\":\"ConnectorPlacement.EquallySpacedRectSide\",\"uuid\":\"2353ed68-b1a1-4775-9ca9-31e268d5443b\"}]},\"type\":\"ConnectorPlacement.EquallySpacedConnector\",\"uuid\":\"d5479f4c-4e65-4791-adcb-73df11f88590\"}],\"packageUris\":[\"http://schema.mathworks.com/mf0/Connector/R2020b\"],\"version\":\"1.0\"}"
  igbt_simple_6 : Subsystem
      settings: PortSchema="{\"entries\":[{\"content\":{\"sides\":[{\"content\":{\"connectorIds\":[\"LConn1\"]},\"type\":\"ConnectorPlacement.EquallySpacedRectSide\",\"uuid\":\"9277da8d-d460-43e6-8478-dd662f15d226\"},{\"content\":{\"connectorIds\":[],\"side\":\"RIGHT\"},\"type\":\"ConnectorPlacement.EquallySpacedRectSide\",\"uuid\":\"a7ece396-f1d9-4f4f-a05b-db1fc65d6e1d\"},{\"content\":{\"connectorIds\":[\"LConn2\"],\"side\":\"TOP\"},\"type\":\"ConnectorPlacement.EquallySpacedRectSide\",\"uuid\":\"fdd70777-e9cf-4317-afb6-cae87f75d5b0\"},{\"content\":{\"connectorIds\":[\"RConn1\"],\"side\":\"BOTTOM\"},\"type\":\"ConnectorPlacement.EquallySpacedRectSide\",\"uuid\":\"2353ed68-b1a1-4775-9ca9-31e268d5443b\"}]},\"type\":\"ConnectorPlacement.EquallySpacedConnector\",\"uuid\":\"d5479f4c-4e65-4791-adcb-73df11f88590\"}],\"packageUris\":[\"http://schema.mathworks.com/mf0/Connector/R2020b\"],\"version\":\"1.0\"}"
  module_1 : Subsystem
  module_2 : Subsystem
  module_3 : Subsystem
  udc(+) : PMIOPort  Side=Left
  u : PMIOPort  Port=2  Side=Right
  v : PMIOPort  Port=3  Side=Right
  udc(-) : PMIOPort  Port=4  Side=Left
  w : PMIOPort  Port=5  Side=Right
  m : Outport
  tag scope: voltage_ee_phase_u=scoped, voltage_ee_phase_v=scoped, voltage_ee_phase_w=scoped
  wires:
  module_3/1(m) -> Bus Creator/3
  module_1/1(m) -> Bus Creator/1
  Bus Creator/1 -> m/1
  module_2/1(m) -> Bus Creator/2
  PS-Simulink Converter2/1 -> [voltage_ee_phase_w]
  PS-Simulink Converter1/1 -> [voltage_ee_phase_v]
  PS-Simulink Converter/1 -> [voltage_ee_phase_u]
  [gate_cmd_Q6] -> Simulink-PS Converter5/1
  [gate_cmd_Q5] -> Simulink-PS Converter4/1
  [gate_cmd_Q3] -> Simulink-PS Converter2/1
  [gate_cmd_Q4] -> Simulink-PS Converter3/1
  [gate_cmd_Q2] -> Simulink-PS Converter1/1
  [gate_cmd_Q1] -> Simulink-PS Converter/1
  gate_commands/1 -> Bus Selector/1
  Bus Selector/6 -> [gate_cmd_Q6]  "<gate_cmd_Q6>"
  Bus Selector/5 -> [gate_cmd_Q5]  "<gate_cmd_Q5>"
  Bus Selector/4 -> [gate_cmd_Q4]  "<gate_cmd_Q4>"
  Bus Selector/3 -> [gate_cmd_Q3]  "<gate_cmd_Q3>"
  Bus Selector/2 -> [gate_cmd_Q2]  "<gate_cmd_Q2>"
  Bus Selector/1 -> [gate_cmd_Q1]  "<gate_cmd_Q1>"
  connections:
  PS-Simulink Converter2/LConn1 -- Voltage Sensor2/RConn1
  PS-Simulink Converter1/LConn1 -- Voltage Sensor1/RConn1
  Voltage Sensor/RConn1 -- PS-Simulink Converter/LConn1
  w/RConn1 -- Voltage Sensor2/LConn1 -- igbt_simple_6/LConn2 -- igbt_simple_5/RConn1
  v/RConn1 -- Voltage Sensor1/LConn1 -- igbt_simple_4/LConn2 -- igbt_simple_3/RConn1
  Voltage Sensor1/RConn2 -- Voltage Sensor2/RConn2 -- Voltage Sensor/RConn2 -- igbt_simple_6/RConn1 -- igbt_simple_4/RConn1 -- igbt_simple_2/RConn1 -- udc(-)/RConn1
  igbt_simple_6/LConn1 -- Simulink-PS Converter5/RConn1
  igbt_simple_5/LConn1 -- Simulink-PS Converter4/RConn1
  igbt_simple_4/LConn1 -- Simulink-PS Converter3/RConn1
  igbt_simple_3/LConn1 -- Simulink-PS Converter2/RConn1
  igbt_simple_2/LConn1 -- Simulink-PS Converter1/RConn1
  igbt_simple_1/LConn1 -- Simulink-PS Converter/RConn1
  udc(+)/RConn1 -- igbt_simple_1/LConn2 -- igbt_simple_5/LConn2 -- igbt_simple_3/LConn2
  u/RConn1 -- Voltage Sensor/LConn1 -- igbt_simple_2/LConn2 -- igbt_simple_1/RConn1

== system afe_dqctrl_inv_psm/inv_dq_mod1/INV_control/inverter_control/Speed control ==
  rotor speed : Inport
  rotor speed ref : Inport  Port=2
  1/Ti : Gain  Gain=psm_ctrl.kp_w  SaturateOnIntegerOverflow=on  OutDataTypeStr=Inherit: Same as input  ParamDataTypeStr=Inherit: Same as input
  Saturation : Saturate  UpperLimit=psm_ctrl.iq_lim  LowerLimit=-psm_ctrl.iq_lim
  Sum1 : Sum  Inputs=+++  SaturateOnIntegerOverflow=on
  Sum2 : Sum  Inputs=-+  SaturateOnIntegerOverflow=on
  Sum3 : Sum  Inputs=-+  SaturateOnIntegerOverflow=on
  Unit Delay4 : UnitDelay  SampleTime=-1
  kp : Gain  Gain=psm_ctrl.ki_w*glb_time.ts_inv  SaturateOnIntegerOverflow=on  OutDataTypeStr=Inherit: Same as input  ParamDataTypeStr=Inherit: Same as input
  torque_ref : Outport
  wires:
  1/Ti/1 -> Sum1/1, Sum3/1
  kp/1 -> Sum1/2
  Sum3/1 -> Unit Delay4/1
  Unit Delay4/1 -> Sum1/3
  rotor speed ref/1 -> Sum2/2
  rotor speed/1 -> Sum2/1
  Sum2/1 -> kp/1, 1/Ti/1
  Sum1/1 -> Saturation/1
  Saturation/1 -> Sum3/2, torque_ref/1

== system afe_dqctrl_inv_psm/inv_dq_mod1/INV_control/inverter_control/current_ctrl ==
  torque_ref : Inport
  Bus Creator1 : BusCreator  Inputs=2
  bemf_observer : Subsystem
  current_ctrl : Subsystem
  current_transformation : Subsystem
  uab : Outport  VectorParamsAs1DForOutWhenUnconnected=off
  wires:
  [ubeta_pu_mod1] -> Bus Creator1/2  "ub"
  [ualpha_pu_mod1] -> Bus Creator1/1  "ua"
  Bus Creator1/1 -> uab/1
  torque_ref/1 -> current_ctrl/1(iq_ref)  "torque_ref"
  [ibeta_pu_mod1] -> bemf_observer/2(ibeta_pu)
  [ialpha_pu_mod1] -> bemf_observer/1(ialpha_pu)
  [ualpha_pu_mod1] -> bemf_observer/3(ualpha_pu)
  [ubeta_pu_mod1] -> bemf_observer/4(ubeta_pu)
  [udcd_pu_inv_mod1] -> current_ctrl/2(udc_pu), bemf_observer/5(udc_pu)

== system afe_dqctrl_inv_psm/inv_dq_mod1/INV_control/inverter_control/encoder-sensorless-switch ==
  Constant : Constant  Value=psm_ctrl.omega_th
  MATLAB Function : MATLAB Function  TreatAsAtomicUnit=on
  Variant Source1 : VariantSource  VariantControls={use_psm_encoder == 1, use_psm_encoder == 0}
  Variant Source2 : VariantSource  VariantControls={use_psm_encoder == 1, use_psm_encoder == 0}
  double_integrator_observer : Subsystem
  omega_pu_psm/hat1 : Scope  NumInputPorts=2
      settings: ActiveDisplayYMinimum=-1  ActiveDisplayYMaximum=1  DataLoggingVariableName=ScopeData13
  phase_elec_psm/hat : Scope  NumInputPorts=2
      settings: ActiveDisplayYMinimum=-1  ActiveDisplayYMaximum=1  DataLoggingVariableName=ScopeData12
  tag scope: motor_phase_ctrl_mod1=scoped, motor_speed_pu_ctrl_mod1=scoped
  wires:
  Variant Source1/1 -> [motor_speed_pu_ctrl_mod1]
  Variant Source2/1 -> [motor_phase_ctrl_mod1]
  [phase_hat_mod1] -> phase_elec_psm/hat/1  "theta_hat_mod1"
  [omega_hat_pu_mod1] -> omega_pu_psm/hat1/1  "omega_hat_pu_mod1"
  [phased_psm] -> double_integrator_observer/1(phase_psm)
  MATLAB Function/1(omega_ctrl) -> Variant Source1/2
  MATLAB Function/2(phase_ctrl) -> Variant Source2/2
  double_integrator_observer/1(phase_psm_hat) -> phase_elec_psm/hat/2, Variant Source2/1, MATLAB Function/1(phase_psm)  "phase_psm_hat"
  double_integrator_observer/2(omega_pu_psm_hat) -> Variant Source1/1, omega_pu_psm/hat1/2, MATLAB Function/2(omega_obs)  "omega_pu_psm_hat"
  [phase_hat_mod1] -> MATLAB Function/3(phase_obs)  "theta_hat_mod1"
  [omega_hat_pu_mod1] -> MATLAB Function/4(omega_psm)  "omega_hat_pu_mod1"
  Constant/1 -> MATLAB Function/5(omega_th)

== system afe_dqctrl_inv_psm/inv_dq_mod1/INV_control/inverter_control/is inv quantizzation and one step delay ==
  is_abc_pu : Inport
  Demux : Demux  Outputs=3
  Mux : Mux  Inputs=3
  is inv quantizzation and one step delay : Subsystem
  isd_abc_pu : Outport
  wires:
  is inv quantizzation and one step delay/2(isd_v_pu) -> Mux/2
  is_abc_pu/1 -> Demux/1
  is inv quantizzation and one step delay/3(isd_w_pu) -> Mux/3
  is inv quantizzation and one step delay/1(isd_u_pu) -> Mux/1
  Demux/1 -> is inv quantizzation and one step delay/1(is_u_pu)
  Mux/1 -> isd_abc_pu/1
  Demux/3 -> is inv quantizzation and one step delay/3(is_w_pu)
  Demux/2 -> is inv quantizzation and one step delay/2(is_v_pu)

== system afe_dqctrl_inv_psm/inv_dq_mod1/INV_control/inverter_control/measurements ==
  Gain : Gain  Gain=psm.psi_bez
  Gain1 : Gain  Gain=psm.psi_bez
  To Workspace10 : ToWorkspace  VariableName=id_pu_sim_mod1  SampleTime=-1
      settings: MaxDataPoints=glb_time.Ns_inv
  To Workspace11 : ToWorkspace  VariableName=iq_pu_sim_mod1  SampleTime=-1
      settings: MaxDataPoints=glb_time.Ns_inv
  To Workspace12 : ToWorkspace  VariableName=uq_pu_sim_mod1  SampleTime=-1
      settings: MaxDataPoints=glb_time.Ns_inv
  To Workspace13 : ToWorkspace  VariableName=iq_pu_ref_sim_mod1  SampleTime=-1
      settings: MaxDataPoints=glb_time.Ns_inv
  To Workspace14 : ToWorkspace  VariableName=id_pu_ref_sim_mod1  SampleTime=-1
      settings: MaxDataPoints=glb_time.Ns_inv
  To Workspace15 : ToWorkspace  VariableName=u_mot_pu_sim_mod1  SampleTime=-1
      settings: MaxDataPoints=glb_time.Ns_inv
  To Workspace2 : ToWorkspace  VariableName=ualpha_pu_sim_mod1  SampleTime=-1
      settings: MaxDataPoints=glb_time.Ns_inv
  To Workspace3 : ToWorkspace  VariableName=ubeta_pu_sim_mod1  SampleTime=-1
      settings: MaxDataPoints=glb_time.Ns_inv
  To Workspace4 : ToWorkspace  VariableName=psi_pu_alpha_hat_sim_mod1  SampleTime=-1
      settings: MaxDataPoints=glb_time.Ns_inv
  To Workspace5 : ToWorkspace  VariableName=psi_pu_beta_hat_sim_mod1  SampleTime=-1
      settings: MaxDataPoints=glb_time.Ns_inv
  To Workspace6 : ToWorkspace  VariableName=psi_r_alpha_hat_sim_mod1  SampleTime=-1
      settings: MaxDataPoints=glb_time.Ns_inv
  To Workspace7 : ToWorkspace  VariableName=ud_pu_sim_mod1  SampleTime=-1
      settings: MaxDataPoints=glb_time.Ns_inv
  To Workspace8 : ToWorkspace  VariableName=psi_r_beta_hat_sim_mod1  SampleTime=-1
      settings: MaxDataPoints=glb_time.Ns_inv
  wires:
  [psi_r_alpha_pu_hat_mod1] -> Gain/1
  [ualpha_pu_mod1] -> To Workspace2/1  "ualpha_pu_mod1"
  Gain/1 -> To Workspace6/1  "psi_r_alpha_hat"
  [psi_r_alpha_pu_hat_mod1] -> To Workspace4/1  "phi_alpha_pu_hat"
  [ubeta_pu_mod1] -> To Workspace3/1  "ubeta_pu_mod1"
  [psi_r_beta_pu_hat_mod1] -> To Workspace5/1  "phi_beta_pu_hat"
  Gain1/1 -> To Workspace8/1  "psi_r_beta_hat"
  [psi_r_beta_pu_hat_mod1] -> Gain1/1
  [u_mot_pu_mod1] -> To Workspace15/1  "u_mot_pu_mod1"
  [iq_pu_ref_mod1] -> To Workspace13/1  "iq_pu_ref_mod1"
  [ud_pu_mod1] -> To Workspace7/1  "ud_pu_mod1"
  [uq_pu_mod1] -> To Workspace12/1  "uq_pu_mod1"
  [iq_pu_mod1] -> To Workspace11/1  "iq_pu_mod1"
  [id_pu_mod1] -> To Workspace10/1  "id_pu_mod1"
  [id_pu_ref_mod1] -> To Workspace14/1  "id_pu_ref_mod1"

== system afe_dqctrl_inv_psm/inv_dq_mod1/INV_control/inverter_control/omega_pu ==
  Abs : Abs  SaturateOnIntegerOverflow=off
  flt : Subsystem
  abs(omega_pu) : Outport
  omega_pu : Outport  Port=2
  wires:
  Abs/1 -> flt/1(input)
  [motor_speed_pu_ctrl_mod1] -> Abs/1, omega_pu/1
  flt/1(output) -> abs(omega_pu)/1

== system afe_dqctrl_inv_psm/inv_dq_mod1/INV_control/inverter_control/phase_acquisition ==
  phase_psm : Inport
  Quantizer : Quantizer  QuantizationInterval=adc_quantization
  Unit Delay : UnitDelay  SampleTime=-1
  Zero-Order Hold : ZeroOrderHold  SampleTime=-1
  phased_psm : Outport
  wires:
  Zero-Order Hold/1 -> Quantizer/1
  Unit Delay/1 -> phased_psm/1
  phase_psm/1 -> Zero-Order Hold/1
  Quantizer/1 -> Unit Delay/1

== system afe_dqctrl_inv_psm/inv_dq_mod1/INV_control/inverter_control/phase_acquisition1 ==
  omega_psm : Inport
  Gain : Gain  Gain=1/psm.omega_bez
  Unit Delay : UnitDelay  SampleTime=-1
  Zero-Order Hold : ZeroOrderHold  SampleTime=-1
  omega_pu_psm : Outport
  wires:
  Zero-Order Hold/1 -> Gain/1
  omega_psm/1 -> Zero-Order Hold/1
  Unit Delay/1 -> omega_pu_psm/1
  Gain/1 -> Unit Delay/1

== system afe_dqctrl_inv_psm/inv_dq_mod1/INV_control/inverter_control/phase_compensation_1 ==
  local_time : Inport
  master_time : Inport  Port=2
  Zero-Order Hold : ZeroOrderHold  SampleTime=-1
  Zero-Order Hold1 : ZeroOrderHold  SampleTime=-1
  alignment_ctrl : Subsystem
  y : Outport
  wires:
  local_time/1 -> Zero-Order Hold/1
  master_time/1 -> Zero-Order Hold1/1
  alignment_ctrl/1(dp) -> y/1
  Zero-Order Hold/1 -> alignment_ctrl/1(local_time)
  Zero-Order Hold1/1 -> alignment_ctrl/2(master_time)

== system afe_dqctrl_inv_psm/inv_dq_mod1/INV_control/inverter_control/space_vector ==
  uab_out : Inport
  Bus Creator : BusCreator  Inputs=3
  Bus Selector : BusSelector  OutputSignals=da,db,dc
  Bus Selector1 : BusSelector  OutputSignals=ua,ub
  C Caller : CCaller  FunctionName=sv_pwm_process_simulink  PortSpecificationStruct="%)30     .    V @   8    (     @         %    \"     4    !     0         %  0 \"0    $    _    07)G3F%M90  4&]R=$YA;64 4V-O<&4     26YD97@     5'EP90      4VEZ90      27-';&]B86P   X    P    !@    @    $          4    (     0    ,    !         !   P!O=70 #@   #     &    \"     0         !0    @    !     P    $         $  # &]U=  .    .     8    (    !          %    \"     $    &     0         0   ...(+2669 chars)"
  Constant : Constant  Value=glb_time.ts_inv
  Constant1 : Constant
  Data Type Conversion1 : DataTypeConversion  OutDataTypeStr=double  SaturateOnIntegerOverflow=off  RndMeth=Floor
  Data Type Conversion15 : DataTypeConversion  OutDataTypeStr=single  SaturateOnIntegerOverflow=off  RndMeth=Floor
  Data Type Conversion16 : DataTypeConversion  OutDataTypeStr=single  SaturateOnIntegerOverflow=off  RndMeth=Floor
  Data Type Conversion17 : DataTypeConversion  OutDataTypeStr=uint32  SaturateOnIntegerOverflow=off  RndMeth=Floor
  Data Type Conversion18 : DataTypeConversion  OutDataTypeStr=single  SaturateOnIntegerOverflow=off  RndMeth=Floor
  Data Type Conversion2 : DataTypeConversion  OutDataTypeStr=double  SaturateOnIntegerOverflow=off  RndMeth=Floor
  Data Type Conversion3 : DataTypeConversion  OutDataTypeStr=double  SaturateOnIntegerOverflow=off  RndMeth=Floor
  Gain1 : Gain  Gain=sqrt(3)/2
  Gain2 : Gain  Gain=sqrt(3)/2
  duvw : Outport
  wires:
  Data Type Conversion15/1 -> C Caller/2
  Bus Selector/2 -> Data Type Conversion2/1  "<db>"
  Data Type Conversion16/1 -> C Caller/3
  Data Type Conversion18/1 -> C Caller/1
  C Caller/1 -> Bus Selector/1
  Bus Creator/1 -> duvw/1
  Data Type Conversion17/1 -> C Caller/4
  Data Type Conversion1/1 -> Bus Creator/1  "du(k)"
  Bus Selector1/2 -> Gain2/1  "<ub>"
  Bus Selector/3 -> Data Type Conversion3/1  "<dc>"
  Bus Selector1/1 -> Gain1/1  "<ua>"
  Data Type Conversion2/1 -> Bus Creator/2  "dv(k)"
  Gain2/1 -> Data Type Conversion15/1
  Bus Selector/1 -> Data Type Conversion1/1  "<da>"
  Gain1/1 -> Data Type Conversion18/1
  Data Type Conversion3/1 -> Bus Creator/3  "dw(k)"
  Constant/1 -> Data Type Conversion16/1
  uab_out/1 -> Bus Selector1/1
  Constant1/1 -> Data Type Conversion17/1

== system afe_dqctrl_inv_psm/inv_dq_mod1/INV_control/inverter_control/speed_reference_generator ==
  Step : Step  Time=time_start_motor_control  FinalValue=omega_m_sim/psm.omega_m_bez
  Step1 : Step  Commented=on  Time=simlength/2  FinalValue=-2*omega_m_sim/omega_m_bez
  Sum : Sum  Inputs=|++
  flt : Subsystem
  omega_ref_pu : Outport
  tag scope: omega_ref_pu_mod1=scoped
  wires:
  Step/1 -> Sum/1
  Step1/1 -> Sum/2
  Sum/1 -> flt/1(input)
  flt/1(output) -> [omega_ref_pu_mod1], omega_ref_pu/1
